simulink model "day26_vehicle_dynamics_model"  (R2026a)
settings: Solver=VariableStepAuto
settings Model: Creator=hem23  LastModifiedBy=hem23

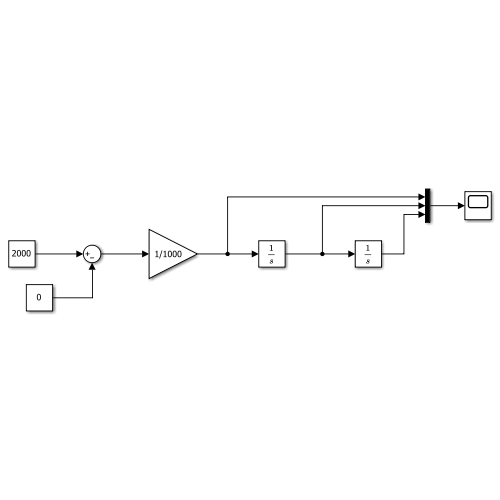
[thumbnail: Simulink's stored preview of the top-level diagram]
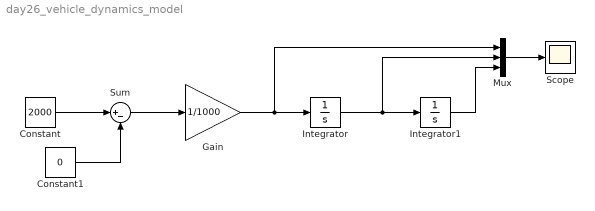
== system day26_vehicle_dynamics_model ==
  Constant : Constant  Value=2000
  Constant1 : Constant  Value=0
  Gain : Gain  Gain=1/1000
  Integrator : Integrator
  Integrator1 : Integrator
  Mux : Mux  Inputs=3
  Scope : Scope
      settings: ActiveDisplayYMinimum=-12.500000000000007  ActiveDisplayYMaximum=112.5000000000001
  Sum : Sum  Inputs=|+-
  wires:
  Constant/1 -> Sum/1
  Sum/1 -> Gain/1
  Gain/1 -> Mux/1, Integrator/1
  Integrator/1 -> Mux/2, Integrator1/1
  Constant1/1 -> Sum/2
  Mux/1 -> Scope/1
  Integrator1/1 -> Mux/3
